simulink model "ball_impact"  (Simulink 8.1)
settings: Solver=ode4  SolverMode=SingleTasking  StartTime=0.0  StopTime=inf  FixedStep=0.0005  RelTol=1e-3
model workspace (MAT data in the model file):
  BKIN_STEP_TIME = 0.0005
  col_x = 1
  col_y = 2
StartFcn:
  |  warndlg('Dexterit-E models cannot run under simulation. Please compile your model and run it from within Dexterit-E.');set_param(bdroot,'SimulationCommand','stop')
undefined symbols (not defined in the file or in its folder): CreateParameterTableGUI, slselsubs
libraries: xpclib x30, simulink x8, KINARM_general x3, KINARM_loads x2, Video x2, KINARM_EP_loads x1
(part 1 of 5)
settings Model: Creator=Supat  LastModifiedBy=Supat  BufferReuse=off
settings DataIOCC: SignalLoggingSaveFormat=Dataset
settings OptimizationCC: BlockReduction=off  OptimizeBlockIOStorage=off  BufferReuse=off  ExpressionFolding=off  ExpressionDepthLimit=128  LocalBlockOutputs=off
settings DebuggingCC: FcnCallInpInsideContextMsg=EnableAllAsError
settings HardwareCC: ProdIntDivRoundTo=Zero  ProdEndianess=LittleEndian  ProdHWDeviceType=Generic->32-bit x86 compatible
settings SFSimCC: SimCustomSourceCode=#include <stdlib.h>
settings RTWCC: SystemTargetFile=xpctarget.tlc  TemplateMakefile=xpc_default_tmf  Description=xPC Target  ProcessScript=xpctarget_make_rtw_hook  CustomSourceCode=#include <stdlib.h>  RTWCompilerOptimization=On
settings CodeAppCC: MaxIdLength=63
settings xpcTargetCC: TargetFcnLib=ansi_tfl_table_tmw.mat  CodeReplacementLibrary=XPC_BLAS  ParMdlRefBuildCompliant=on  ConcurrentExecutionCompliant=on  CombineSignalStateStructs=off  MATLABClassNameForMDSCustomization=xpcAperiodicCustomization  GRTInterface=on  GenerateAllocFcn=off  xPCTaskExecutionProfile=off  xPCRL32EventNumber=5000  xPCisDownloadable=off  xPCLoadParamSetFile=off  xPCConcurrentTasks=off  xPCEnableSFAnimation=off

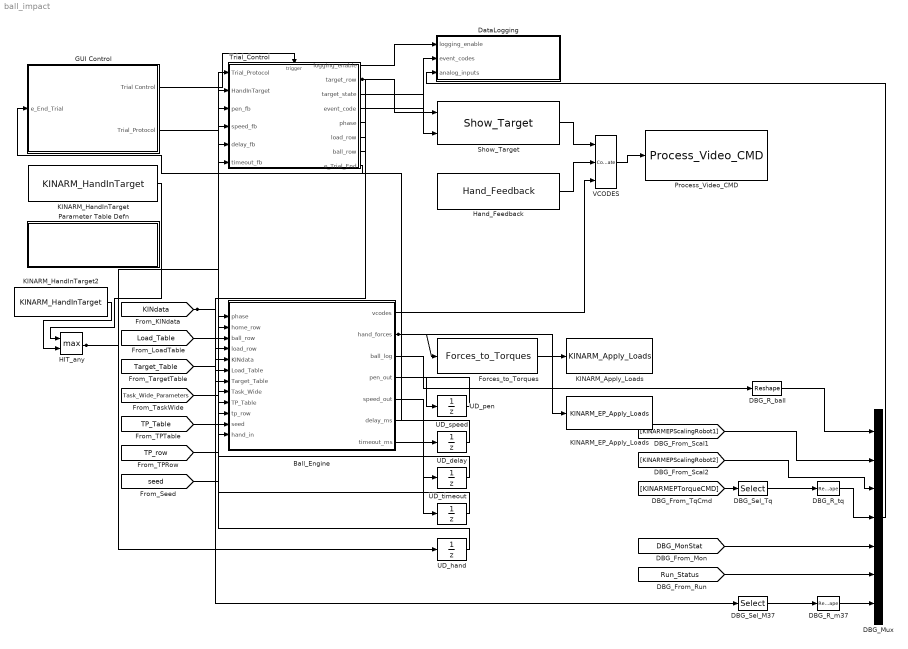
== system ball_impact ==
  Ball_Engine : MATLAB Function  TreatAsAtomicUnit=on  SystemSampleTime=0.001
  DBG_Mux : Mux  Inputs=7
  DBG_R_ball : Reshape
  DBG_R_m37 : Reshape
  DBG_R_tq : Reshape
  DBG_Sel_M37 : Selector  NumberOfDimensions=2  IndexOptions=Index vector (dialog),Index vector (dialog)  Indices=[1 2],37  OutputSizes=1
  DBG_Sel_Tq : Selector  InputPortWidth=4  IndexOptions=Index vector (dialog)  Indices=[1 2]  OutputSizes=1
  DataLogging : Subsystem  mask(DataLogging){log_event_codes=on, log_analog_inputs=on}
      mask prompts: log_event_codes "Log event codes"; log_analog_inputs "Log analog inputs"
      mask help:
      | <b>Do not rename this block, it must be called 'DataLogging'.</b>
      | <p>
      | This block collects data and event codes and transfers them to the GUI.
      | <p>
      | This block must be present in all task programs.
      mask init:
      | %this stops us from running a simulation
      | set_param(bdroot,'StartFcn',' warndlg(''Dexterit-E models cannot run under simulation. Please compile your model and run it from within Dexterit-E.'');set_param(bdroot,''SimulationCommand'',''stop'')')
      | 
      | block_path = gcb;  % store block path, as gcb may change with block operations
      |  
      | idxs = findstr(block_path, '/DataLogging');
      | [idxCount, n] = size(idxs);
      | [m, strlen] = size(block_path);
      | bColorSet = 0;
      | 
      | dexcheck();
      | if idxCount == 0 || idxs(1) ~= strlen - 11
      |     fprintf('=========ERROR====================\n');
      |     fprintf('%s should be called DataLogging, attempting to rename.\n', block_path);
      |     try
      |         set_param(block_path, 'Name', 'DataLogging');
      |         block_path = gcb;  % store block path, as gcb may change with block operations
      |         fprintf('Rename successful\n');
      |     catch err
      |         fprintf('Rename failed. You may have 2 DataLogging blocks or another improperly named block.\n');
      |        	set_param(block_path, 'BackgroundColor', '[0.9, 0, 0]');
      |         bColorSet = 1;
      |     end
      |     fprintf('=============================\n');
      | end
      | 
      | log_event_codes = strcmp(get_param(block_path, 'log_event_codes'), 'on');
      | log_analog_inputs = strcmp(get_param(block_path, 'log_analog_inputs'), 'on');
      | 
      | % Handle the event codes setting: swap the 'Event Codes' inport with a constant block or 
      | % vice versa, if necessary, so that it matches the setting.
      | block_type = get_param([block_path '/event_codes'], 'BlockType');
      |  
      | if log_event_codes && ~strcmp(block_type, 'Inport') || ...  % if a change is required...
      |    ~log_event_codes && strcmp(block_type, 'Inport')
      |     
      |     % ...delete the existing block, ...
      |     pos = get_param([block_path '/event_codes'], 'Position');
      |     delete_line(block_path, 'event_codes/1', 'Create Event Codes Subsystem/1');
      |     delete_block([block_path '/event_codes']);
      |     
      |     % ...add an Inport or a 0-value Constant in place of the previous block (according to
      |     % the new setting), update the signal width flag, and then...
      |     if log_event_codes && ~strcmp(block_type, 'Inport')
      |         add_block('built-in/Inport', [block_path '/event_codes'], 'Name', 'event_codes');
      |         set_param([block_path '/Create Event Codes Subsystem/Not Logging Event Codes'], 'Value', '0');
      |     else
      |         add_block('built-in/Constant', [block_path '/event_codes'], 'Name', 'event_codes');
      |         set_param([block_path '/event_codes'], 'Value', '0');
      |         set_param([block_path '/Create Event Codes Subsystem/Not Logging Event Codes'], 'Value', '1');
      |     end
      |     
      |     % ...connect the new block.
      |     set_param([block_path '/event_codes'], 'Position', pos);
      |     add_line(block_path, 'event_codes/1', 'Create Event Codes Subsystem/1');
      | end
      | 
      | % Swap the 'analog_data' inport with a constant block or vice versa according to the corresponding setting.
      | block_type = get_param([block_path '/analog_inputs'], 'BlockType');
      | 
      | if log_analog_inputs && ~strcmp(block_type, 'Inport') || ...  % if a change is required...
      |    ~log_analog_inputs && strcmp(block_type, 'Inport')
      |     
      |     % ...delete the existing block, ...
      |     pos = get_param([block_path '/analog_inputs'], 'Position');
      |     delete_line(block_path, 'analog_inputs/1', 'Create Analog Inputs Subsystem/1');
      |     delete_block([block_path '/analog_inputs']);
      |     
      |     % ...add an Inport or a 0-value Constant in place of the previous block (according to
      |     % the new setting), update the signal width flag, and then...
      |     if log_analog_inputs && ~strcmp(block_type, 'Inport')
      |         add_block('built-in/Inport', [block_path '/analog_inputs'], 'Name', 'analog_inputs');
      |         set_param([block_path '/Create Analog Inputs Subsystem/Not Logging Analog Inputs'], 'Value', '0');
      |     else
      |         add_block('built-in/Constant', [block_path '/analog_inputs'], 'Name', 'analog_inputs');
      |         set_param([block_path '/analog_inputs'], 'Value', '0');
      |         set_param([block_path '/Create Analog Inputs Subsystem/Not Logging Analog Inputs'], 'Value', '1');
      |     end
      |     
      |     % ...connect the new block.
      |     set_param([block_path '/analog_inputs'], 'Position', pos);
      |     add_line(block_path, 'analog_inputs/1', 'Create Analog Inputs Subsystem/1');
      | end
      | 
      | % Create the text label for the block, and use it to create the first in a 
      | % list of drawing commands that will be used to draw the mask icon.
      | label = 'Logging:\n ';
      |  
      | if log_event_codes
      |    label = [label 'Event codes\n'];
      | end
      |  
      | label = [label 'KINARM data\n'];
      |     
      | if log_analog_inputs
      |     label = [label 'Analog inputs\n'];
      | end
      | 
      | draw_commands = 'disp(label); ';
      | 
      | % Ensure the inports appear in a fixed order, and for each inport found add
      | % to the list of drawing commands a command to label it.
      | inports = find_system(block_path, 'LookUnderMasks', 'all', 'FollowLinks', 'on', 'SearchDepth', 1, 'BlockType', 'Inport');
      | 
      | for i = 1:length(inports)
      |     inport_name = char(get_param(inports(i), 'Name'));
      |     
      |     if strcmp(inport_name, 'logging_enable')
      |         port = '1';
      |     elseif strcmp(inport_name, 'event_codes')
      |         port = '2';
      |     elseif strcmp(inport_name, 'analog_inputs') && log_event_codes
      |         port = '3';
      |     elseif strcmp(inport_name, 'analog_inputs')
      |         port = '2';
      |     end
      |     
      |     set_param([block_path '/' inport_name], 'Port', port);
      |     draw_commands = [draw_commands 'port_label(''input'', ' port ', ''' inport_name '''); '];
      | end
      | 
      | % Apply the drawing commands.
      | set_param(block_path, 'MaskDisplay', draw_commands);
      | 
      | %%% Handle background colours if link status changes.  
      | checkBackgroundColour(block_path, 'General');
      | 
      | % For gaze tracking, the packet length is variable, so we need to check off that option the Receive UDP block.
      | % But that option is only availabe starting in R2010a. The TDK is presently created/maintained using R2007b so
      | % if the MATLAB version is >= R2010a, then we need to check this option
      | current_ver = ver('MATLAB');
      | current_ver_parts = sscanf(current_ver.Version, '%d.%d.%d')';
      | if length(current_ver_parts) < 3
      |     current_ver_parts(3) = 0;
      | end
      | 
      | desired_ver = '7.10.0';
      | desired_ver_parts = sscanf(desired_ver, '%d.%d.%d')';
      | if length(desired_ver_parts) < 3
      |     desired_ver_parts(3) = 0;
      | end
      | 
      | if (sign(current_ver_parts - desired_ver_parts) * [1; 0.1; 0.01]) >= 0
      | 	set_param([block_path '/Receive_Gaze/Receive'], 'vblLen', 'on')
      | end
      mask Help:
      | Sends data and event codes to the GUI.
      | 
      | <H2>Library </H2>
      | General
      | 
      | <H2>Description </H2>
      | <b>Do not rename this block, it must be called 'DataLogging'.</b>
      | <p>
      | The DataLogging block collects data and event codes and sends it to the GUI for saving.  It also passes on Task Program information that is invisible to the user, and so must be present even if no data is going to be saved.
      | <P>
      | <B><I>This block must be present in all Task Programs, even if no data is going to be saved.</I></B>
      | 
      | 
      | <H2>Parameters and Dialog Box</H2>
      | <B>Log event codes: </B> checking this parameter causes the GUI to log event codes specified by the event_codes input.
      | <P>
      | <B>Log analog inputs: </B> checking this parameter causes the GUI to log analog data specified by the analog_inputs input.
      | <P>
      | <B>analog_inputs: </B> this vector input specifies the data from analog inputs and other arbitrary data to be logged by the GUI.
      | <P>
      | <B>event_codes: </B> this input should be a vector of 16 bit integers.  It is passed on to the GUI, which saves the integers as event codes (i.e. they are timestamped so that events that occurred duing a task can be related to the other saved data).
      | <P>
      | <B>logging_enable: </B> this input is used by the GUI to indicate when to save data.  When logging_enable is 1, data is saved.  When logging_enable is 0, data is not saved.  (Note: data saving is also affected by the Run/Pause button in the GUI.  When the task is paused, data is no longer saved regardless of the value of this input).
      mask Display: disp(label); port_label('input', 1, 'logging_enable'); port_label('input', 2, 'event_codes'); port_label('input', 3, 'analog_inputs');
  Forces_to_Torques : KINARM_loads/Forces_to_Torques
  GUI Control : Subsystem  mask(GUI Control){target_type_str=Circle, Target_Type=1, XYcols=[0 0], Vcols=3, Lcols=4, indices_padding=[0 0 0 0;0 0 0 0], task_version=1.0, show_repeat_trial_flag=off}
      mask prompts: target_type_str "Target Type"; Target_Type "Target Type (Int)"; XYcols "Columns for X and Y Position"; Vcols "Column(s) for Visual Target Attributes"; Lcols "Column(s) for Logical Target Attributes"; indices_padding "Indices Padding"; task_version "Task version"; show_repeat_trial_flag "Show repeat trial flag input"
      mask help:
      | <b>Do not rename this block, it must be called 'GUI Control'.</b>
      | <p>
      | This block allows the GUI to control the Task Program.  In particular, the order and control of trials is implemented via this block.
      | <p>
      | This block also defines the target preview information to show the user on the GUI, i.e. the display of greyed-out versions of all visual targets defined in the Task Protocol, as well as the display of the "logical" versions of the targets used for hand-in-target calculations.  In order for the GUI to show this target information for a task, the columns of the target table that define the positions and visual and logical characteristics of targets need to be specified here.
      mask init:
      | % Check the version of MATLAB that is being used, using logic from Mathworks' R12-
      | % backwards-compatible verLessThan function. More information can be found at:
      | %
      | % http://www.mathworks.com/support/solutions/data/1-38LI61.html?solution=1-38LI61
      | %
      | % If the MATLAB version is R2007b (7.5) or higher, include the s-function used to 
      | % disable SMIs on startup. This prevents needless CPU overload errors.
      | performBKINModelSetup();
      | 
      | current_ver = ver('MATLAB');
      | current_ver_parts = sscanf(current_ver.Version, '%d.%d.%d')';
      | if length(current_ver_parts) < 3
      |     current_ver_parts(3) = 0;
      | end
      | 
      | desired_ver = '7.5.0';
      | desired_ver_parts = sscanf(desired_ver, '%d.%d.%d')';
      | if length(desired_ver_parts) < 3
      |     desired_ver_parts(3) = 0;
      | end
      | 
      | result = (sign(current_ver_parts - desired_ver_parts) * [1; 0.1; 0.01]) < 0;
      | 
      | current_block_path = gcb;
      | pos = get_param([current_block_path '/ICH7'], 'Position');
      | block_type = get_param([current_block_path '/ICH7'], 'BlockType');
      | 
      | idxs = findstr(current_block_path, '/GUI Control');
      | [idxCount, n] = size(idxs);
      | [m, strlen] = size(current_block_path);
      | bColorSet = 0;
      | if idxCount == 0 || idxs(1) ~= strlen - 11
      |     fprintf('=========ERROR====================\n');
      |     fprintf('%s should be called GUI Control, attempting to rename.\n', current_block_path);
      |     try
      |         set_param(current_block_path, 'Name', 'GUI Control');
      |         current_block_path = gcb;
      |         fprintf('Rename successful\n');
      |     catch err
      |         fprintf('Rename failed. You may have 2 GUI Control blocks or another improperly named block.\n');
      |        	set_param(current_block_path, 'BackgroundColor', '[0.9, 0, 0]');
      |         bColorSet = 1;
      |     end
      |     fprintf('=============================\n');
      | end
      | 
      | 
      | if result
      |     % The MATLAB version is less than 7.5, so the s-function should be removed if present. 
      |     if ~strcmp(block_type, 'Constant')
      |         delete_block([current_block_path '/ICH7']);
      |         add_block('built-in/Constant', [current_block_path '/ICH7'], 'Name', 'ICH7');
      |         set_param([current_block_path '/ICH7'], 'Position', pos);
      |         set_param([current_block_path '/ICH7'], 'Value', '0');
      |     end
      | else
      | 	% The MATLAB version is 7.5 or higher, so the s-function should be added if not already there.
      |     %if ~strcmp(block_type, 'S-Function')
      |         delete_block([current_block_path '/ICH7']);
      |         add_block('built-in/S-Function', [current_block_path '/ICH7'], 'Name', 'ICH7');
      |         set_param([current_block_path '/ICH7'], 'Position', pos);
      |         set_param([current_block_path '/ICH7'], 'FunctionName', 'ich10');
      |     %end
      | end
      | 
      | % Record the xPC Target version in a Constant block for reference by the Dexterit-E GUI.
      | v = ver;
      | 
      | for i=1:length(v)
      |     if strcmp(v(i).Name, 'xPC Target')
      |         set_param([current_block_path '/xPC Version'], 'Value', v(i).Version);
      |     end
      | end
      |  
      | % Record the current time (i.e. compile time) in a Constant block for reference by the Dexterit-E GUI.
      | set_param([current_block_path '/dlm build time'], 'Value', num2str(now,20));
      | 
      | % Handle the 'Show repeat trial flag input' setting: swap the flag input with a constant block or
      | % vice versa in accordance with the setting (.
      | show_repeat_trial_flag = strcmp(get_param(current_block_path, 'show_repeat_trial_flag'), 'on');
      | block_type = get_param([current_block_path '/Repeat_Trial_Flag'], 'BlockType');
      | 
      | if show_repeat_trial_flag && ~strcmp(block_type, 'Inport') || ...  % if a change is required...
      |    ~show_repeat_trial_flag && strcmp(block_type, 'Inport')
      |     
      |     % ...delete the existing block, ...
      |     pos = get_param([current_block_path '/Repeat_Trial_Flag'], 'Position');
      |     delete_line(current_block_path, 'Repeat_Trial_Flag/1', 'Task Execution Control Subsystem/1');
      |     delete_block([current_block_path '/Repeat_Trial_Flag']);
      |     
      |     % ...add an Inport or a 0-value Constant in place of the previous block (according to
      |     % the new setting), update the signal width flag, and then...
      |     if show_repeat_trial_flag && ~strcmp(block_type, 'Inport')
      |         add_block('built-in/Inport', [current_block_path '/Repeat_Trial_Flag'], 'Name', 'Repeat_Trial_Flag');
      |     else
      |         add_block('built-in/Constant', [current_block_path '/Repeat_Trial_Flag'], 'Name', 'Repeat_Trial_Flag');
      |         set_param([current_block_path '/Repeat_Trial_Flag'], 'Value', '0');
      |     end
      |     
      |     % ...connect the new block.
      |     set_param([current_block_path '/Repeat_Trial_Flag'], 'Position', pos);
      |     add_line(current_block_path, 'Repeat_Trial_Flag/1', 'Task Execution Control Subsystem/1');
      | end
      | 
      | %after correcting the number of columns, redo the column grabbing
      | target_type_str=get_param(current_block_path, 'target_type_str');
      | XY_text=get_param(current_block_path, 'XYcols');
      | V_text=get_param(current_block_path, 'Vcols');
      | L_text=get_param(current_block_path, 'Lcols');
      | 
      | columntext=strvcat('Target Visualization in GUI', ' ', target_type_str,['X, Y columns: ', XY_text], ['Visual attribute column(s): ', V_text],['Logical attribute column(s): ', L_text]);
      | 
      | % Create the text label for the block.
      | draw_commands = 'disp(columntext); ';
      | 
      | inports = find_system(current_block_path, 'LookUnderMasks', 'all', 'FollowLinks', 'on', 'SearchDepth', 1, 'BlockType', 'Inport');
      | 
      | for i = 1:length(inports)
      |     inport_name = char(get_param(inports(i), 'Name'));
      |     
      |     if strcmp(inport_name, 'Repeat_Trial_Flag')
      |         set_param([current_block_path '/Repeat_Trial_Flag'], 'Port', '1');
      |     end
      |     
      |     draw_commands = [draw_commands 'port_label(''input'', ' int2str(i) ', ''' inport_name '''); '];
      | end
      | 
      | outports = find_system(current_block_path, 'LookUnderMasks', 'all', 'FollowLinks', 'on', 'SearchDepth', 1, 'BlockType', 'Outport');
      | 
      | for i = 1:length(outports)
      |     outport_name = char(get_param(outports(i), 'Name'));
      |     draw_commands = [draw_commands 'port_label(''output'', ' int2str(i) ', ''' outport_name '''); '];
      | end
      | 
      | set_param(current_block_path, 'MaskDisplay', draw_commands);
      | 
      | block_path = gcb;  % store block path, as gcb may change with block operations
      | 
      | %%% Handle background colours if link status changes.  
      | checkBackgroundColour(block_path, 'General');
      mask Help:
      | Used by the GUI to control the Task Program
      | 
      | <H2>Library </H2>
      | General
      | 
      | <H2>Description </H2>
      | <b>Do not rename this block, it must be called 'GUI Control'.</b>
      | <p>
      | This block allows the GUI to control the Task Program. In particular, the order and control of trials is implemented through the use of this block.
      | <P>
      | This block also tells the GUI which preview target information to show the user (i.e. greyed-out display of all targets in the Task Protocol). In order for the GUI to show target information for a task, the correct columns in the target table need to be specified in the dialog box (see below).
      | <P>
      | There are 2 inputs to this block:
      | <P>
      | <B>Repeat_Trial_Flag: </B> this scalar input is examined by the GUI Control block at the end of a trial to determine if the trial that just finished should be repeated. If it is greater than 0 <i>and</i> if the GUI has requested to "repeat error trials", then the trial just finished will be added to a repeat block that will commence at the end of the present block.  If this input equals 0 <i>or</i> if the GUI has requested not to "repeat error trials", then the trial will not be queued for repetition.
      | <P>
      | <B>e_End_Trial:</B> this event input is used to indicate that a trial has finished. It should be an event from a Stateflow chart that is created upon completion of a trial. Upon this event occuring (which occurs on both rising and falling edge), the outputs of this block will change to reflect the next trial's outputs.
      | <P>
      | There are 2 outputs from this block:
      | <P>
      | <B>Trial_Control: </B> this event output is used to control the stateflow chart in the Task Program.  There are 2 events muxed together in this output: a 1 kHz clock and an end-trial-now event.  The clock is a true 1 kHz clock in that it is 0.5 ms high, 0.5 ms low (i.e. it should trigger an event in the subsquent flowchart to which it is attached on ONLY the rising edge).  The clock only runs when the GUI has commanded the Task Program to run (i.e. when the GUI commands a pause to the Task Program, this clock stops executing).  The end-trial-now event triggers an event on both the rising and falling edges.   It is triggered by the GUI and pressing of the Pause button in the GUI when certain conditions apply - these conditions include when the Pause option is: Skip Trial, Repeat Trial Now or Repeat Trial Later.  Those options in the GUI assume that the end-trial-now event has been used in the Task Program such that it will cause an immediate exit of the trial.  Please see the Customing Task Programs documentation for more details.
      | <P>
      | <B>Trial_Protocol</B> this vector output contains the row from the Trial Protocol Table corresponding to the present trial.  It is typically connected to the stateflow chart to implement trial-specfic behavior.
      | <P>
      | <B><I>This block must be present in all Task Programs.</I></B>
      | 
      | <H2>Parameters and Dialog Box</H2>
      | <P>The GUI is capable of showing greyed-out versions of all targets in a target table for the user to have a quick view of all targets in the task protocol.  Similarly, the GUI can also show outlined versions of all the the 'logical' targets (the targets used for hand-in-target calculations) in the task protocol.
      | <P>
      | <B>Target Type:</B> the type of preview target to display.
      | <P>
      | <B>Columns for X and Y Position:</B> the columns in the Target Table used to define the x and y positions.
      | <P>
      | <B>Column(s) for Visual Target Attributes:</B>: the columns that specify the visual characteristics of a target that are specific to that type of target. These are similar to the target type-specific columns specified in the Show_Target block.
      | <P><I>Circle:</I> radius of the circle (cm).
      | <P><I>Ellipse:</I> major radius (cm), minor radius (cm), rotation angle (degrees).  If no rotation is desired, the rotation column index should be set to 0.
      | <P><I>Rectangle:</I> length (cm), height (cm), rotation angle (degrees).  If no rotation is desired, the rotation column index should be set to 0.
      | <P><I>Line:</I> end point x-axis position relative to start point (cm), end point y-axis position relative to start point (cm), width (cm).
      | <P><I>Triangle:</I> length (cm), height (cm), offset of peak of triangle relative to midpoint of the length (cm), rotation angle (degrees). If a height column index of 0 is specified, then an equilateral triangle with sides of the specified length is used.  If no rotation is desired, the rotation column index should be set to 0.
      | <P>
      | <B>Column(s) for Logical Target Attributes:</B>: The columns that specify the logical characteristics (used to determine if the hand is in a target or not) of a target that are specific to that type of target. They are of the same format as the visual characteristics for each target, and can be the same as those columns or different. They are only relevant if using the HandInTarget block. If not using that block, enter 0 for each logical target attribute column.
      | <P>
      mask TypeOptions target_type_str: Circle | Ellipse | Rectangle | Line | Triangle
      mask Callback target_type_str:
      | target_type_str=get_param(gcb, 'target_type_str');
      | XYcols=[str2num(get_param(gcb, 'XYcols')) 0 0];
      | Vcols=[str2num(get_param(gcb, 'Vcols')) 0 0 0 0 0 0];
      | Lcols=[str2num(get_param(gcb, 'Lcols')) 0 0 0 0 0 0];
      | 
      | switch target_type_str(1:3)
      | 	case 'Cir'
      | 		numcol=1;
      |         set_param(gcb, 'Target_Type', '1');
      | 	case 'Ell'
      | 		numcol=3;
      |         set_param(gcb, 'Target_Type', '2');
      |     case 'Rec'
      |         numcol=3;
      |         set_param(gcb, 'Target_Type', '3');
      |     case 'Lin'
      |         numcol=3;
      |         set_param(gcb, 'Target_Type', '4');
      |     case 'Tri'
      |         numcol=4;
      |         set_param(gcb, 'Target_Type', '5');
      |     otherwise
      | 		numcol=1;
      |         set_param(gcb, 'Target_Type', '1');
      | end
      | 
      | set_param(gcb, 'XYcols', mat2str(XYcols(1:2)));
      | set_param(gcb, 'Vcols', mat2str(Vcols(1:numcol)));
      | set_param(gcb, 'Lcols', mat2str(Lcols(1:numcol)));
      | 
      | indices_padding=zeros(2,5);
      | set_param(gcb, 'indices_padding', mat2str(indices_padding(:, 1:(5-numcol))));
      mask Display: disp(columntext); port_label('input', 1, 'e_End_Trial'); port_label('output', 1, 'Trial Control'); port_label('output', 2, 'Trial_Protocol');
  HIT_any : MinMax  Function=max  Inputs=2  SaturateOnIntegerOverflow=on  InputSameDT=on
  Hand_Feedback : KINARM_general/Hand_Feedback  feedback_cntl_src=none
  KINARM_Apply_Loads : KINARM_loads/KINARM_Apply_Loads  up_duration=500  down_duration=500  max_torque=12
  KINARM_EP_Apply_Loads : KINARM_EP_loads/KINARM_EP_Apply_Loads  up_duration=500  down_duration=500  max_force=30
  KINARM_HandInTarget : KINARM_general/KINARM_HandInTarget  use_dominant_hand=on  target_type=Circle  num_states=1  attribcol1=[4]  attribcol2=[3]  attribcol3=[3]  attribcol4=[3]  attribcol5=[0]
  KINARM_HandInTarget2 : KINARM_general/KINARM_HandInTarget  use_dominant_hand=off  target_type=Circle  num_states=1  attribcol1=[4]  attribcol2=[3]  attribcol3=[3]  attribcol4=[3]  attribcol5=[0]
  Parameter Table Defn : Subsystem  LoadFcn=|  InitFcn=CreateParameterTableGUI('init')  mask{ShowInLibBrowser=0}
      | CreateParameterTableGUI('load')                                                        
      | % only put a pattern on the icon for R2013a and later, because prior versions of MATALB
      | % do not properly support transparency for mask icons                                  
      | current_ver = ver('MATLAB');                                                           
      | current_ver_parts = sscanf(current_ver.Version, '%d.%d.%d')';                          
      | if length(current_ver_parts) < 3                                                       
      |     current_ver_parts(3) = 0;                                                          
      | end                                                                                    
      | desired_ver = '8.1.0';		% This is the base version for MATLAB                          
      | desired_ver_parts = sscanf(desired_ver, '%d.%d.%d')';                                  
      | if length(desired_ver_parts) < 3                                                       
      |     desired_ver_parts(3) = 0;                                                          
      | end                                                                                    
      | show_icon = (sign(current_ver_parts - desired_ver_parts) * [1; 0.1; 0.01]) >= 0;       
      | if show_icon                                                                           
      | 	set_param(gcb, 'MaskDisplay', 'image(''ParameterTableDefnIcon.png'')' );              
      | else                                                                                   
      |   set_param(gcb, 'MaskDisplay', '' );                                                  
      | end
      mask prompts: ShowInLibBrowser "Mask Parameter 1:"
      mask init:
      | % NOTE: the ShowInLibBrowser Parameter for this mask is required by Simulink in order
      | % for this block to appear in the Library Browser because the OpenFcn callback is defined
      | % for this block.  For some reason, when the OpenFcn callback is defined, Simulink does NOT 
      | % show the block in the Library Browser.  The requirement of the "ShowInLibBrowser appears 
      | % to be some sort of hack solution provided by Mathworks, but it works.
      | 
      | edit_parameters_blockpath = gcb;
      | 
      | %%% Handle background colours if link status changes.  
      | checkBackgroundColour(edit_parameters_blockpath, 'General');
      | 
      | % all data used by the mask is passed to it through the UserData parameter
      | % the UserData is only available because we set UserDataPersistent to 'on' in the m-file
      | all_tab_data = get_param(edit_parameters_blockpath, 'UserData');
      | 
      | % only make the changes if required.  The update/build process is not compatible with deleting of blocks, etc.
      | % so the apply flag is only set if the dialog has been opened and changes need to be applied OR if the model 
      | % has just been loaded
      | if all_tab_data(1).apply
      | 	% delete all sub-blocks to ensure a clean empty block
      | 	Simulink.SubSystem.deleteContents(edit_parameters_blockpath);
      | 
      | 	number_tabs = length(all_tab_data);
      | 
      | 	for tab = 1:number_tabs
      | 		% Add one sub-block per tab, to contain the various constants blocks
      | 		block_pos = [100, -40, 240, 0] + tab * [0 60 0 60];
      | 		sub_block_name = all_tab_data(tab).sub_block_name;
      | 		block_path = [edit_parameters_blockpath '/' sub_block_name];
      | 
      | 		add_block('built-in/Subsystem', block_path,  'Position', mat2str(block_pos) );
      | 
      | 		% Add new constant blocks for each row to the "tab" block (i.e. each parameter gets its own constant block)
      | 		for row_index = 1:all_tab_data(tab).num_param
      | 			% Add a constant sub-block to the Parameter Table block, for use by Dex
      | 			curr_param = all_tab_data(tab).params(row_index);
      | 			current_path = [edit_parameters_blockpath '/' sub_block_name];
      | 			block_pos = [200, -40, 240, 0] + row_index * [0 60 0 60];
      | 			blockname = curr_param.blockname;
      | 			block_path = [current_path '/' blockname];
      | 			add_block('built-in/Constant', block_path, 'Value', curr_param.paramindex, 'Position', mat2str(block_pos) );
      | 			% Add a terminator
      | 			block_pos = block_pos + [100 10 100 -10];
      | 			terminator_name = ['Terminator' num2str(row_index)];
      | 			terminator_path = [current_path '/' terminator_name];
      | 			add_block('built-in/Terminator', terminator_path, 'Position', mat2str(block_pos));
      | 			% connect the constant and terminator blocks
      | 			add_line(current_path, [blockname '/1'], [terminator_name '/1']);
      | 		end
      | 	end
      | 	all_tab_data(1).apply = false;
      | 	set_param(edit_parameters_blockpath, 'UserData', all_tab_data);
      | end
      | 	
      | 
      | % % % % only put a pattern on the icon for R2013a and later, because prior versions of MATALB
      | % % % % do not properly support transparency for mask icons
      | % % % 
      | % % % current_ver = ver('MATLAB');
      | % % % current_ver_parts = sscanf(current_ver.Version, '%d.%d.%d')';
      | % % % if length(current_ver_parts) < 3
      | % % %     current_ver_parts(3) = 0;
      | % % % end
      | % % % 
      | % % % desired_ver = '8.1.0';		% This is the base version for MATLAB
      | % % % desired_ver_parts = sscanf(desired_ver, '%d.%d.%d')';
      | % % % if length(desired_ver_parts) < 3
      | % % %     desired_ver_parts(3) = 0;
      | % % % end
      | % % % 
      | % % % show_icon = (sign(current_ver_parts - desired_ver_parts) * [1; 0.1; 0.01]) >= 0;
      | % % % 
      | % % % if show_icon
      | % % % 	set_param(edit_parameters_blockpath, 'MaskDisplay', 'image(''test3.png'')' );
      | % % % else
      | % % % 	set_param(edit_parameters_blockpath, 'MaskDisplay', '' );
      | % % % end
      settings: CopyFcn=CreateParameterTableGUI('copy')  OpenFcn=CreateParameterTableGUI('open')
      mask Display: image('ParameterTableDefnIcon.png')
  Process_Video_CMD : Video/Process_Video_CMD
  Show_Target : Video/Show_Target  target_type=Circle  num_states=2  attribcol1=[5 5 0 3]  attribcol2=[6 6 0 3]  attribcol3=[0 0 0 0]  attribcol4=[0 0 0 0]  attribcol5=[0 0 24 0]  stateindices_padding=[0 0 0 0 0 0 0;0 0 0 0 0 0 0;0 0 0 0 0 0 0;0 0 0 0 0 0 0;0 0 0 0 0 0 0]  source=dialog  opacity=100  target_display=Both subject and operator displays  num_col=4
  Trial_Control : Stateflow chart  TreatAsAtomicUnit=on
  UD_delay : UnitDelay  SampleTime=0.001
  UD_hand : UnitDelay  SampleTime=0.001
  UD_pen : UnitDelay  SampleTime=0.001
  UD_speed : UnitDelay  SampleTime=0.001
  UD_timeout : UnitDelay  SampleTime=0.001
  VCODES : Concatenate  NumInputs=3  Mode=Multidimensional array
  wires:
  GUI Control/1(Trial Control) -> Trial_Control/Trigger
  GUI Control/2(Trial_Protocol) -> Trial_Control/1(Trial_Protocol)
  KINARM_HandInTarget/1 -> HIT_any/1
  KINARM_HandInTarget2/1 -> HIT_any/2
  HIT_any/1 -> Trial_Control/2(HandInTarget), UD_hand/1
  UD_pen/1 -> Trial_Control/3(pen_fb)
  UD_speed/1 -> Trial_Control/4(speed_fb)
  UD_delay/1 -> Trial_Control/5(delay_fb)
  UD_timeout/1 -> Trial_Control/6(timeout_fb)
  Trial_Control/1(logging_enable) -> DataLogging/1(logging_enable)
  Trial_Control/2(target_row) -> Show_Target/1, Ball_Engine/2(home_row)
  Trial_Control/3(target_state) -> Show_Target/2
  Trial_Control/4(event_code) -> DataLogging/2(event_codes)
  Trial_Control/5(phase) -> Ball_Engine/1(phase)
  Trial_Control/6(load_row) -> Ball_Engine/4(load_row)
  Trial_Control/7(ball_row) -> Ball_Engine/3(ball_row)
  Trial_Control/8(e_Trial_End) -> GUI Control/1(e_End_Trial)
  [KINdata] -> Ball_Engine/5(KINdata), DBG_Sel_M37/1
  [Load_Table] -> Ball_Engine/6(Load_Table)
  [Target_Table] -> Ball_Engine/7(Target_Table)
  [Task_Wide_Parameters] -> Ball_Engine/8(Task_Wide)
  [TP_Table] -> Ball_Engine/9(TP_Table)
  [TP_row] -> Ball_Engine/10(tp_row)
  [seed] -> Ball_Engine/11(seed)
  UD_hand/1 -> Ball_Engine/12(hand_in)
  Show_Target/1 -> VCODES/1
  Hand_Feedback/1 -> VCODES/2
  Ball_Engine/1(vcodes) -> VCODES/3
  VCODES/1 -> Process_Video_CMD/1
  Ball_Engine/2(hand_forces) -> Forces_to_Torques/1, KINARM_EP_Apply_Loads/1
  Forces_to_Torques/1 -> KINARM_Apply_Loads/1
  Ball_Engine/4(pen_out) -> UD_pen/1
  Ball_Engine/5(speed_out) -> UD_speed/1
  Ball_Engine/6(delay_ms) -> UD_delay/1
  Ball_Engine/7(timeout_ms) -> UD_timeout/1
  Ball_Engine/3(ball_log) -> DBG_R_ball/1
  DBG_R_ball/1 -> DBG_Mux/1
  [KINARMEPScalingRobot1] -> DBG_Mux/2
  [KINARMEPScalingRobot2] -> DBG_Mux/3
  [KINARMEPTorqueCMD] -> DBG_Sel_Tq/1
  DBG_Sel_Tq/1 -> DBG_R_tq/1
  DBG_R_tq/1 -> DBG_Mux/4
  [DBG_MonStat] -> DBG_Mux/5
  [Run_Status] -> DBG_Mux/6
  DBG_Sel_M37/1 -> DBG_R_m37/1
  DBG_R_m37/1 -> DBG_Mux/7
  DBG_Mux/1 -> DataLogging/3(analog_inputs)

== system ball_impact/DataLogging ==
  note: Section 5: User-specified data.
  note: Note: for data which is at the user's option to include, e.g. event codes, some extra work is done to ensure that the user
      | does not have to observe warnings about unconnected inputs during a build if they turn off those inputs in the mask. When
      | one of these inputs is turned off, the corresponding inport is replaced with a Constant that gives the frame's number-of-items
      | count (e.g. "Number of Event Codes" in the event code subsystem) a value of 0, even though the frame will still contain a
      | single "dummy" value because the signal still exists and must have at least one element by definition. Clients examining the
      | data frames must be aware of this and ignore the dummy value.
      |
      | If a user opts to keep the inport available but connects nothing to it, Simulink resolves that as a single signal with value 0.
  note: Section 3: KINARM data. KINARM data consists of segment
      | position, velocity and acceleration, as well as subject pointer /
      | fingertip position, motor torque, and force sensor data for all arms.
      | KINARM data is currently required in all tasks.
  note: Section 2: User event codes.
  note: Section 1: State information common to all tasks.
  note: Section 4: User-specified analog input data.
  note: This block assembles individual data frames, which are collected into packets and sent out by the network transfer subsystem.
      |
      | Data frames may consist of up to 300 floating point values, that is, the network transfer subsystem can accept an input of up
      | to 300 values wide. However, the number of values available to the user of this block is less than 300, as each data frame
      | must include information about task state common to all tasks. The frame can be considered as consisting of a number of
      | "sections" of data shown below, with section one containing the common state information.
  logging_enable : Inport
  event_codes : Inport  Port=2
  analog_inputs : Inport  Port=3
  Create Analog Inputs Subsystem : Subsystem
  Create Custom Data Subsystem : Subsystem
  Create Event Codes Subsystem : Subsystem
  Create KINARM Data Subsystem : Subsystem
  Create Task State Subsystem : Subsystem
  Keep alive : Subsystem
  Mux : Mux  Inputs=5
  Mux1 : Mux  Inputs=2
  Network Transfer Subsystem : Subsystem
  Poll Force Plates : Subsystem
  Poll KINARM : Subsystem
      mask init:
      | block_path = gcb;  % store block path, as gcb may change with block operations
      | 
      | % Handle background colours if link status changes.  If the link is resolved, 
      | % make the block back to the library colour.  If the link is not resolved, 
      | % change the colour to something other than the library block colour (but 
      | % only change it if it is the library colour, that way end-users can choose
      | % their own colour.
      | link_status = get_param(block_path, 'LinkStatus');
      | block_parent = get_param(block_path, 'Parent');
      | set_param(block_path, 'BackgroundColor', '[1, 1, 1]');
      | 
      | % Handle KINARM Exo Torques
      | 
      | % Find out if the KINARMTorqueCMD Goto block exists elsewhere in the Simulink model.
      | gotoblock = find_system(bdroot, 'LookUnderMasks', 'all', 'FollowLinks', 'on', 'BlockType', 'Goto');
      | goto_exists = 0;
      | 
      | for i = 1:length(gotoblock)
      |     if strcmp(get_param(char(gotoblock(i)), 'GotoTag'), 'KINARMTorqueCMD')
      |         goto_exists = 1;
      |     end
      | end
      | 
      | % Check whether a From block with the name KINARMTorqueCMD exists in the current block.
      | fromblock = find_system(gcb, 'LookUnderMasks', 'all', 'FollowLinks', 'on', 'SearchDepth', 1, 'BlockType', 'From');
      | from_exists = 0;
      | 
      | for i = 1:length(fromblock)
      |     if strcmp(get_param(char(fromblock(i)), 'GotoTag'), 'KINARMTorqueCMD')
      |         from_exists = 1;
      |     end
      | end
      | 
      | if from_exists == goto_exists
      |     % Do nothing if either both the From and Goto exist or if neither exists.
      | 
      | elseif goto_exists == 1 && from_exists == 0
      |     % If a >From is not paired with an existing Goto, delete the Constant block and make the From block.
      |     pos = get_param([gcb '/ZeroTorque'], 'position');
      | 
      |     delete_line(gcb, 'ZeroTorque/1', 'AddTorques/1');
      |     delete_block([gcb '/ZeroTorque']);
      | 
      |     add_block('built-in/From', [gcb '/TorqueCMD']);
      |     set_param([gcb '/TorqueCMD'], 'position', pos);
      |     add_line(gcb, 'TorqueCMD/1', 'AddTorques/1');
      |     set_param([gcb '/TorqueCMD'], 'GotoTag', 'KINARMTorqueCMD');
      | 
      | else
      |     % If a From block exists but the Goto is missing, delete the From block and replace it with a Constant.
      |     pos = get_param([gcb '/TorqueCMD'], 'position');
      | 
      |     delete_line(gcb, 'TorqueCMD/1', 'AddTorques/1');
      |     delete_block([gcb '/TorqueCMD']);
      | 
      |     add_block('built-in/Constant', [gcb '/ZeroTorque']);
      |     set_param([gcb '/ZeroTorque'], 'position', pos);
      |     add_line(gcb, 'ZeroTorque/1', 'AddTorques/1');
      |     set_param([gcb '/ZeroTorque'], 'Value', '[0 0 0 0]');
      | end
      | 
      | 
      | % Handle KINARM EP Torques
      | 
      | % Find out if the KINARMEPTorqueCMD Goto block exists elsewhere in the Simulink model.
      | gotoblock = find_system(bdroot, 'LookUnderMasks', 'all', 'FollowLinks', 'on', 'BlockType', 'Goto');
      | goto_exists = 0;
      | 
      | for i = 1:length(gotoblock)
      |     if strcmp(get_param(char(gotoblock(i)), 'GotoTag'), 'KINARMEPTorqueCMD')
      |         goto_exists = 1;
      |     end
      | end
      | 
      | % Check whether a From block with the name KINARMTorqueCMD exists in the current block.
      | fromblock = find_system(gcb, 'LookUnderMasks', 'all', 'FollowLinks', 'on', 'SearchDepth', 1, 'BlockType', 'From');
      | from_exists = 0;
      | 
      | for i = 1:length(fromblock)
      |     if strcmp(get_param(char(fromblock(i)), 'GotoTag'), 'KINARMEPTorqueCMD')
      |         from_exists = 1;
      |     end
      | end
      | 
      | if from_exists == goto_exists
      |     % Do nothing if either both the >From and Goto exist or if neither exists.
      | 
      | elseif goto_exists == 1 && from_exists == 0
      |     % If a From is not paired with an existing Goto, delete the Constant block and make the From block.
      |     pos = get_param([gcb '/ZeroEPTorque'], 'position');
      | 
      |     delete_line(gcb, 'ZeroEPTorque/1', 'AddTorques/2');
      |     delete_block([gcb '/ZeroEPTorque']);
      | 
      |     add_block('built-in/From', [gcb '/EPTorqueCMD']);
      |     set_param([gcb '/EPTorqueCMD'], 'position', pos);
      |     add_line(gcb, 'EPTorqueCMD/1', 'AddTorques/2');
      |     set_param([gcb '/EPTorqueCMD'], 'GotoTag', 'KINARMEPTorqueCMD');
      | 
      | else
      |     % If a From block exists but the Goto is missing, delete the From block and replace it with a Constant.
      |     pos = get_param([gcb '/EPTorqueCMD'], 'position');
      | 
      |     delete_line(gcb, 'EPTorqueCMD/1', 'AddTorques/2');
      |     delete_block([gcb '/EPTorqueCMD']);
      | 
      |     add_block('built-in/Constant', [gcb '/ZeroEPTorque']);
      |     set_param([gcb '/ZeroEPTorque'], 'position', pos);
      |     add_line(gcb, 'ZeroEPTorque/1', 'AddTorques/2');
      |     set_param([gcb '/ZeroEPTorque'], 'Value', '[0 0 0 0]');
      | end
  Receive_Gaze : Subsystem
  custom_version : Constant  Value=3  OutDataTypeStr=uint32
  wires:
  Create Custom Data Subsystem/1(Out1) -> Mux/5
  Create Analog Inputs Subsystem/1(Out1) -> Mux/4
  Create KINARM Data Subsystem/1(Out1) -> Mux/3
  Create Event Codes Subsystem/1(Out1) -> Mux/2
  Create Task State Subsystem/1(Out1) -> Mux/1
  logging_enable/1 -> Create Task State Subsystem/1(In1)
  [KINdata] -> Create Task State Subsystem/2(In2), Create KINARM Data Subsystem/1(In1)
  Mux/1 -> Network Transfer Subsystem/1(data_frame)
  custom_version/1 -> Mux1/1
  [status_data] -> Mux1/2
  Mux1/1 -> Create Custom Data Subsystem/1(In1)
  event_codes/1 -> Create Event Codes Subsystem/1(In1)
  analog_inputs/1 -> Create Analog Inputs Subsystem/1(In1)
